simulink model "ex_5"  (R2025a)
settings: Solver=ode4  StartTime=0.0  StopTime=10  FixedStep=0.01  RelTol=1e-3  EnableMultiTasking=on
settings Model: Creator=Lukasz  LastModifiedBy=Anna Witkowska
settings SolverCC: AlgebraicLoopSolver=TrustRegion
settings DataIOCC: LimitDataPoints=on  SaveFormat=Array  SignalLoggingSaveFormat=ModelDataLogs  ReturnWorkspaceOutputs=off  SignalLoggingName=sigsOut
settings OptimizationCC: ExpressionDepthLimit=2147483647.0  LifeSpan=inf
settings DebuggingCC: SaveWithParameterizedLinksMsg=none  UnderspecifiedInitializationDetection=Classic  MergeDetectMultiDrivingBlocksExec=none  SignalResolutionControl=TryResolveAllWithWarning  MultiTaskDSMMsg=warning  MultiTaskCondExecSysMsg=none  UnconnectedInputMsg=warning  UnconnectedOutputMsg=warning  UnconnectedLineMsg=warning  StateNameClashWarn=warning  SFUnexpectedBacktrackingDiag=warning  SFNoUnconditionalDefaultTransitionDiag=warning  SFExecutionAtInitializationDiag=none  ArithmeticOperatorsInVariantConditions=warning
settings HardwareCC: ProdBitPerPointer=32.0  ProdBitPerSizeT=32.0  ProdBitPerPtrDiffT=32.0  ProdLargestAtomicFloat=None  ProdIntDivRoundTo=Undefined  ProdEndianess=Unspecified  ProdWordSize=32.0  ProdHWDeviceType=32-bit Generic  TargetUnknown=on
settings ModelReferenceCC: EnableRefExpFcnMdlSchedulingChecks=on  PropagateSignalLabelsOutOfModel=off
settings SFSimCC: SimUseLocalCustomCode=off  CustomCodeUndefinedFunction=UseInterfaceOnly
settings RTWCC: RTWUseLocalCustomCode=off  GPUComputeCapability=3.5
settings CodeAppCC: StateflowObjectComments=on
settings GRTTargetCC: TargetLangStandard=C89/C90 (ANSI)  CombineOutputUpdateFcns=off  GRTInterface=on
settings ConfigComp: CovMetricSettings=dw  CovSaveCumulativeToWorkspaceVar=on  CovSaveSingleToWorkspaceVar=on  CovExternalEMLEnable=off

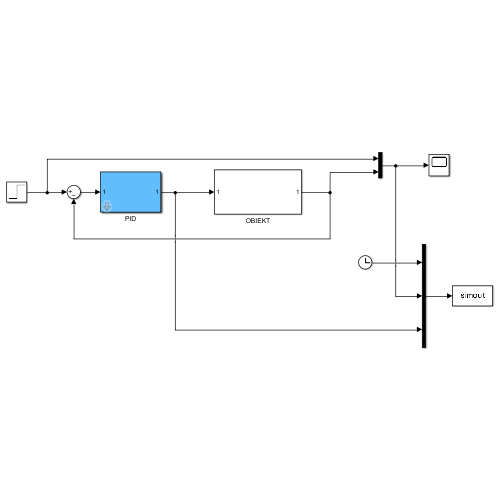
[thumbnail: Simulink's stored preview of the top-level diagram]
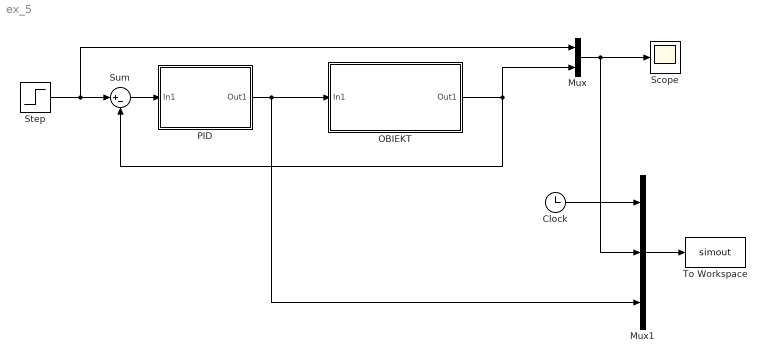
== system ex_5 ==
  Clock : Clock
  Mux : Mux  Inputs=2
  Mux1 : Mux  Inputs=3
  OBIEKT : Subsystem
  PID : Subsystem  mask{Kp=3.5484, Kd=1.5583, Ki=9.5782}
      mask prompts: Kp "Kp - wzmocnienie proporcjalne"; Kd "Kd - czas wyprzedzenia"
  Scope : Scope
      settings: ActiveDisplayYMinimum=2.5  ActiveDisplayYMaximum=42.5
  Step : Step  SampleTime=0
  Sum : Sum  Inputs=|+-  SaturateOnIntegerOverflow=on
  To Workspace : ToWorkspace  VariableName=simout  SaveFormat=Array  SampleTime=-1
  wires:
  Mux/1 -> Mux1/2, Scope/1
  Mux1/1 -> To Workspace/1
  Clock/1 -> Mux1/1
  PID/1(Out1) -> Mux1/3, OBIEKT/1(In1)
  Step/1 -> Sum/1, Mux/1
  Sum/1 -> PID/1(In1)
  OBIEKT/1(Out1) -> Sum/2, Mux/2

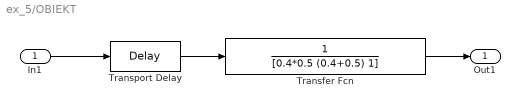
== system ex_5/OBIEKT ==
  In1 : Inport
  Transfer Fcn : TransferFcn  Denominator=[0.4*0.5 (0.4+0.5) 1]
  Transport Delay : TransportDelay  DelayTime=0.2
  Out1 : Outport
  wires:
  Transfer Fcn/1 -> Out1/1
  In1/1 -> Transport Delay/1
  Transport Delay/1 -> Transfer Fcn/1

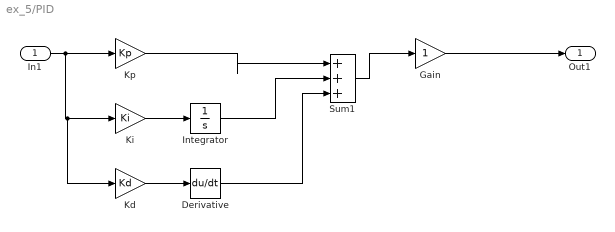
== system ex_5/PID ==
  In1 : Inport
  Derivative : Derivative
  Gain : Gain  SaturateOnIntegerOverflow=on  OutDataTypeStr=Inherit: Same as input  ParamDataTypeStr=Inherit: Same as input
  Integrator : Integrator
  Kd : Gain  Gain=Kd  SaturateOnIntegerOverflow=on  OutDataTypeStr=Inherit: Same as input  ParamDataTypeStr=Inherit: Same as input
  Ki : Gain  Gain=Ki
  Kp : Gain  Gain=Kp  SaturateOnIntegerOverflow=on  OutDataTypeStr=Inherit: Same as input  ParamDataTypeStr=Inherit: Same as input
  Sum1 : Sum  Inputs=|+++  SaturateOnIntegerOverflow=on
  Out1 : Outport
  wires:
  In1/1 -> Kd/1, Ki/1, Kp/1
  Kp/1 -> Sum1/1
  Gain/1 -> Out1/1
  Sum1/1 -> Gain/1
  Ki/1 -> Integrator/1
  Integrator/1 -> Sum1/2
  Derivative/1 -> Sum1/3
  Kd/1 -> Derivative/1
